simulink model "F2026_ECE597_01_Closed_Loop_Step_Response_PID"  (R2025a)
settings: Solver=VariableStepAuto  StartTime=0.0  StopTime=60.0  RelTol=1e-3
values from neighbouring files (symbols this model uses):
  A = [[-0.59 0.92 0.61 -9.82]; [-0.23 -6.31 4.42 0.19]; [ 0.78 -5.59 -5.92 0]; [0 0 1 0]]    [F2026_ECE597_01_Closed_Loop_Step_Response_PID_Driver.m]
  B = B_w_wind(:,1:2)    [F2026_ECE597_01_Closed_Loop_Step_Response_PID_Driver.m]
  C = [[1 0 0 0]; [0 0 0 1]]    [F2026_ECE597_01_Closed_Loop_Step_Response_PID_Driver.m]
  D = zeros(2, 2)    [F2026_ECE597_01_Closed_Loop_Step_Response_PID_Driver.m]
  delta_airspeed = target_airspeed - airspeed_init    (= 2.1)    [F2026_ECE597_01_Closed_Loop_Step_Response_PID_Driver.m]
  delta_pitch = target_pitch - pitch_init    [F2026_ECE597_01_Closed_Loop_Step_Response_PID_Driver.m]
  elevator_max = deg2rad(20) - elevator_init    [F2026_ECE597_01_Closed_Loop_Step_Response_PID_Driver.m]
  elevator_min = -deg2rad(20) - elevator_init    [F2026_ECE597_01_Closed_Loop_Step_Response_PID_Driver.m]
  G_Airspeed = 1.0    (= 1)    [F2026_ECE597_01_Closed_Loop_Step_Response_PID_Driver.m]
  G_Decoupler = [0.019614 -0.005618; 0.036387 0.501756]    [F2026_ECE597_01_Closed_Loop_Step_Response_PID_Driver.m]
  G_Pitch_Angle = 1.0    (= 1)    [F2026_ECE597_01_Closed_Loop_Step_Response_PID_Driver.m]
  kD_1 = 0.43    [F2026_ECE597_01_Closed_Loop_Step_Response_PID_Driver.m]
  kD_2 = 1.04    [F2026_ECE597_01_Closed_Loop_Step_Response_PID_Driver.m]
  kI_1 = 1.54    [F2026_ECE597_01_Closed_Loop_Step_Response_PID_Driver.m]
  kI_2 = 1.46    [F2026_ECE597_01_Closed_Loop_Step_Response_PID_Driver.m]
  kP_1 = 0.98    [F2026_ECE597_01_Closed_Loop_Step_Response_PID_Driver.m]
  kP_2 = 2.97    [F2026_ECE597_01_Closed_Loop_Step_Response_PID_Driver.m]
  throttle_max = 1.0 - throttle_init    (= 0.56)    [F2026_ECE597_01_Closed_Loop_Step_Response_PID_Driver.m]
  throttle_min = 0.0 - throttle_init    (= -0.44)    [F2026_ECE597_01_Closed_Loop_Step_Response_PID_Driver.m]
libraries: slpidlib x2
settings Model: Creator=gresham2  LastModifiedBy=gresham2

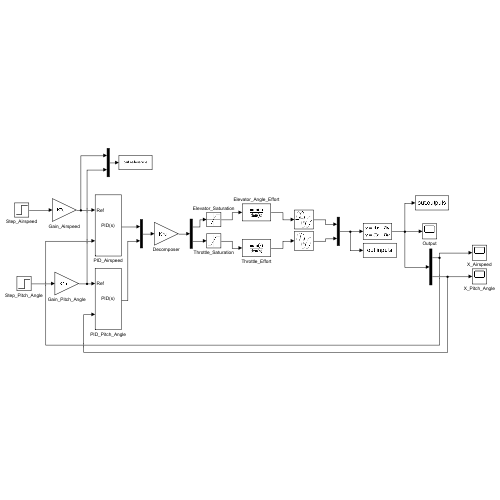
[thumbnail: Simulink's stored preview of the top-level diagram]
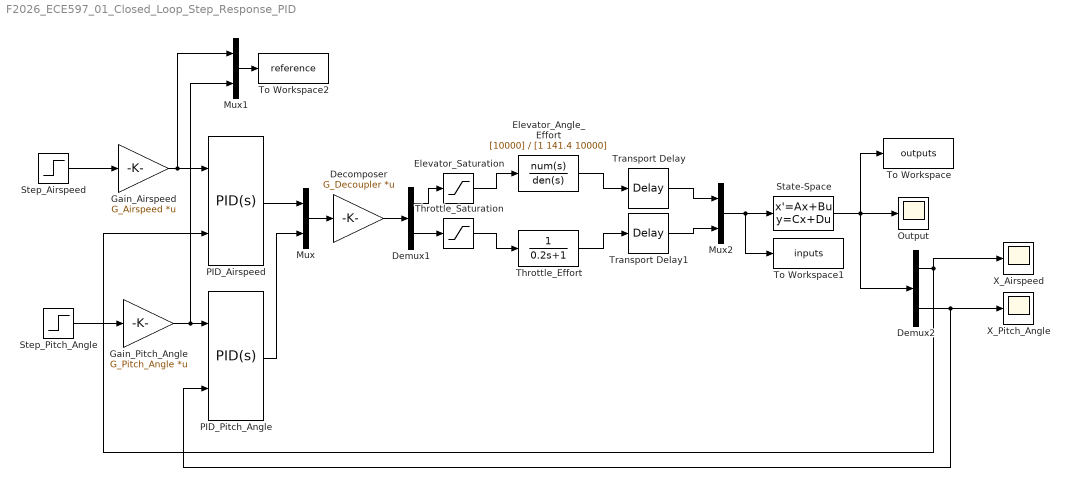
== system F2026_ECE597_01_Closed_Loop_Step_Response_PID ==
  Decomposer : Gain  Gain=G_Decoupler  Multiplication=Matrix(K*u)
  Demux1 : Demux  Outputs=2
  Demux2 : Demux  Outputs=2
  Elevator_Angle_Effort : TransferFcn  Numerator=[10000]  Denominator=[1 141.4 10000]
  Elevator_Saturation : Saturate  UpperLimit=elevator_max  LowerLimit=elevator_min
  Gain_Airspeed : Gain  Gain=G_Airspeed  Multiplication=Matrix(K*u)
  Gain_Pitch_Angle : Gain  Gain=G_Pitch_Angle  Multiplication=Matrix(K*u)
  Mux : Mux  Inputs=2
  Mux1 : Mux  Inputs=2
  Mux2 : Mux  Inputs=2
  Output : Scope
      settings: ActiveDisplayYMinimum=-1  ActiveDisplayYMaximum=1
  PID_Airspeed : slpidlib/PID Controller (2DOF)  Controller=PID  Form=Parallel  TimeDomain=Continuous-time  UseExternalTs=off  SampleTime=-1  IntegratorMethod=Forward Euler  FilterMethod=Forward Euler  ControllerParametersSource=internal  P=kP_1  I=kI_1  UseKiTs=off  D=kD_1  UseExternalDerivativeSource=off  N=100  UseFilter=on  b=1.0  c=0.0  TunerSelectOption=Transfer Function Based (PID Tuner App)  InitialConditionSource=internal  InitialConditionForIntegrator=0  InitialConditionForFilter=0  DifferentiatorICPrevScaledInput=0  ExternalReset=none  TrackingMode=off  Kt=1  LimitOutput=off  SatLimitsSource=internal  UpperSaturationLimit=inf  LowerSaturationLimit=-inf  LinearizeAsGain=on  AntiWindupMode=none  Kb=1  LimitIntegrator=off  UpperIntegratorSaturationLimit=inf  LowerIntegratorSaturationLimit=-inf  POutMin=[]  POutMax=[]  IOutMin=[]  IOutMax=[]  DOutMin=[]  DOutMax=[]  NOutMin=[]  NOutMax=[]  bOutMin=[]  bOutMax=[]  cOutMin=[]  cOutMax=[]  SumOutMin=[]  SumOutMax=[]  SaturationOutMin=[]  SaturationOutMax=[]  PParamMin=[]  PParamMax=[]  IParamMin=[]  IParamMax=[]  DParamMin=[]  DParamMax=[]  NParamMin=[]  NParamMax=[]  bParamMin=[]  bParamMax=[]  cParamMin=[]  cParamMax=[]  KbParamMin=[]  KbParamMax=[]  KtParamMin=[]  KtParamMax=[]  KbOutMin=[]  KbOutMax=[]  KtOutMin=[]  KtOutMax=[]  IntegratorOutMin=[]  IntegratorOutMax=[]  FilterOutMin=[]  FilterOutMax=[]  SumI1OutMin=[]  SumI1OutMax=[]  SumI2OutMin=[]  SumI2OutMax=[]  SumI3OutMin=[]  SumI3OutMax=[]  SumI4OutMin=[]  SumI4OutMax=[]  SumDOutMin=[]  SumDOutMax=[]  Sum1OutMin=[]  Sum1OutMax=[]  Sum2OutMin=[]  Sum2OutMax=[]  Sum3OutMin=[]  Sum3OutMax=[]  DifferentiatorOutMin=[]  DifferentiatorOutMax=[]  FilterDiffOutCoefMin=[]  FilterDiffOutCoefMax=[]  ReciprocalOutMin=[]  ReciprocalOutMax=[]  SumDenOutMin=[]  SumDenOutMax=[]  SumNumOutMin=[]  SumNumOutMax=[]  DivideOutMin=[]  DivideOutMax=[]  UdiffTsProdOutMin=[]  UdiffTsProdOutMax=[]  NTsProdOutMin=[]  NTsProdOutMax=[]  UintegralTsProdOutMin=[]  UintegralTsProdOutMax=[]  UngainTsProdOutMin=[]  UngainTsProdOutMax=[]  ClampingZeroOutDataTypeStr=Inherit: Inherit via back propagation  ClampingZeroOutMin=[]  ClampingZeroOutMax=[]  FilterDenConstantOutDataTypeStr=Inherit: Inherit via back propagation  FilterDenConstantOutMin=[]  FilterDenConstantOutMax=[]  PCopyOutDataTypeStr=Inherit: Inherit via back propagation  PCopyOutMin=[]  PCopyOutMax=[]  NCopyOutDataTypeStr=Inherit: Inherit via back propagation  NCopyOutMin=[]  NCopyOutMax=[]  IntegratorContinuousStateAttributes=''  IntegratorStateMustResolveToSignalObject=off  IntegratorRTWStateStorageClass=Auto  FilterContinuousStateAttributes=''  FilterStateMustResolveToSignalObject=off  FilterRTWStateStorageClass=Auto  ParallelPVariant=InternalParameters  IdealPVariant=Disabled  IVariant=InternalParameters  DVariant=InternalParameters  bVariant=InternalParameters  cVariant=InternalParameters  IntegratorVariant=Continuous  SatVariant=Disabled  AWVariant=Passthrough  PCopyVariant=Disabled  TRVariant=Disabled  FdbkBlocksVariant=Forward  IdealPFdbkVariant=Disabled  SatFdbkVariant=Disabled  DerivativeFilterVariant=ContFilter  NVariant=InternalParameters  NCopyVariant=Disabled  FilterICVariant=InternalICsFilter  IntegratorICVariant=InternalICs  ExternalResetVariant=Disabled  TRSumVariant=Passthrough  SumFdbkVariant=Disabled  SumVariant=Sum_PID  TsampFilterVariant=InternalTs  TsampNgainVariant=Passthrough  TsampIntegralVariant=Disabled_SignalSpec  ExternalSaturationOutDataTypeStr=Inherit: Same as second input  DerivativeSourceVariant=ErrorSignal  PreIntVariant=InternalPreInt
  PID_Pitch_Angle : slpidlib/PID Controller (2DOF)  Controller=PID  Form=Parallel  TimeDomain=Continuous-time  UseExternalTs=off  SampleTime=-1  IntegratorMethod=Forward Euler  FilterMethod=Forward Euler  ControllerParametersSource=internal  P=kP_2  I=kI_2  UseKiTs=off  D=kD_2  UseExternalDerivativeSource=off  N=100  UseFilter=on  b=1.0  c=0.0  TunerSelectOption=Transfer Function Based (PID Tuner App)  InitialConditionSource=internal  InitialConditionForIntegrator=0  InitialConditionForFilter=0  DifferentiatorICPrevScaledInput=0  ExternalReset=none  TrackingMode=off  Kt=1  LimitOutput=off  SatLimitsSource=internal  UpperSaturationLimit=inf  LowerSaturationLimit=-inf  LinearizeAsGain=on  AntiWindupMode=none  Kb=1  LimitIntegrator=off  UpperIntegratorSaturationLimit=inf  LowerIntegratorSaturationLimit=-inf  POutMin=[]  POutMax=[]  IOutMin=[]  IOutMax=[]  DOutMin=[]  DOutMax=[]  NOutMin=[]  NOutMax=[]  bOutMin=[]  bOutMax=[]  cOutMin=[]  cOutMax=[]  SumOutMin=[]  SumOutMax=[]  SaturationOutMin=[]  SaturationOutMax=[]  PParamMin=[]  PParamMax=[]  IParamMin=[]  IParamMax=[]  DParamMin=[]  DParamMax=[]  NParamMin=[]  NParamMax=[]  bParamMin=[]  bParamMax=[]  cParamMin=[]  cParamMax=[]  KbParamMin=[]  KbParamMax=[]  KtParamMin=[]  KtParamMax=[]  KbOutMin=[]  KbOutMax=[]  KtOutMin=[]  KtOutMax=[]  IntegratorOutMin=[]  IntegratorOutMax=[]  FilterOutMin=[]  FilterOutMax=[]  SumI1OutMin=[]  SumI1OutMax=[]  SumI2OutMin=[]  SumI2OutMax=[]  SumI3OutMin=[]  SumI3OutMax=[]  SumI4OutMin=[]  SumI4OutMax=[]  SumDOutMin=[]  SumDOutMax=[]  Sum1OutMin=[]  Sum1OutMax=[]  Sum2OutMin=[]  Sum2OutMax=[]  Sum3OutMin=[]  Sum3OutMax=[]  DifferentiatorOutMin=[]  DifferentiatorOutMax=[]  FilterDiffOutCoefMin=[]  FilterDiffOutCoefMax=[]  ReciprocalOutMin=[]  ReciprocalOutMax=[]  SumDenOutMin=[]  SumDenOutMax=[]  SumNumOutMin=[]  SumNumOutMax=[]  DivideOutMin=[]  DivideOutMax=[]  UdiffTsProdOutMin=[]  UdiffTsProdOutMax=[]  NTsProdOutMin=[]  NTsProdOutMax=[]  UintegralTsProdOutMin=[]  UintegralTsProdOutMax=[]  UngainTsProdOutMin=[]  UngainTsProdOutMax=[]  ClampingZeroOutDataTypeStr=Inherit: Inherit via back propagation  ClampingZeroOutMin=[]  ClampingZeroOutMax=[]  FilterDenConstantOutDataTypeStr=Inherit: Inherit via back propagation  FilterDenConstantOutMin=[]  FilterDenConstantOutMax=[]  PCopyOutDataTypeStr=Inherit: Inherit via back propagation  PCopyOutMin=[]  PCopyOutMax=[]  NCopyOutDataTypeStr=Inherit: Inherit via back propagation  NCopyOutMin=[]  NCopyOutMax=[]  IntegratorContinuousStateAttributes=''  IntegratorStateMustResolveToSignalObject=off  IntegratorRTWStateStorageClass=Auto  FilterContinuousStateAttributes=''  FilterStateMustResolveToSignalObject=off  FilterRTWStateStorageClass=Auto  ParallelPVariant=InternalParameters  IdealPVariant=Disabled  IVariant=InternalParameters  DVariant=InternalParameters  bVariant=InternalParameters  cVariant=InternalParameters  IntegratorVariant=Continuous  SatVariant=Disabled  AWVariant=Passthrough  PCopyVariant=Disabled  TRVariant=Disabled  FdbkBlocksVariant=Forward  IdealPFdbkVariant=Disabled  SatFdbkVariant=Disabled  DerivativeFilterVariant=ContFilter  NVariant=InternalParameters  NCopyVariant=Disabled  FilterICVariant=InternalICsFilter  IntegratorICVariant=InternalICs  ExternalResetVariant=Disabled  TRSumVariant=Passthrough  SumFdbkVariant=Disabled  SumVariant=Sum_PID  TsampFilterVariant=InternalTs  TsampNgainVariant=Passthrough  TsampIntegralVariant=Disabled_SignalSpec  ExternalSaturationOutDataTypeStr=Inherit: Same as second input  DerivativeSourceVariant=ErrorSignal  PreIntVariant=InternalPreInt
  State-Space : StateSpace  A=A  B=B  C=C  D=D  InitialCondition=0
  Step_Airspeed : Step  After=delta_airspeed  SampleTime=0
  Step_Pitch_Angle : Step  After=delta_pitch  SampleTime=0
  Throttle_Effort : TransferFcn  Denominator=[0.2 1]
  Throttle_Saturation : Saturate  UpperLimit=throttle_max  LowerLimit=throttle_min
  To Workspace : ToWorkspace  VariableName=outputs  SaveFormat=Timeseries  SampleTime=-1
  To Workspace1 : ToWorkspace  VariableName=inputs  SaveFormat=Timeseries  SampleTime=-1
  To Workspace2 : ToWorkspace  VariableName=reference  SaveFormat=Timeseries  SampleTime=-1
  Transport Delay : TransportDelay  DelayTime=0.07
  Transport Delay1 : TransportDelay  DelayTime=0.05
  X_Airspeed : Scope
      settings: ActiveDisplayYMinimum=-1  ActiveDisplayYMaximum=1  DataLoggingVariableName=ScopeData4
  X_Pitch_Angle : Scope
      settings: ActiveDisplayYMinimum=-1  ActiveDisplayYMaximum=1  DataLoggingVariableName=ScopeData3
  wires:
  State-Space/1 -> To Workspace/1, Output/1, Demux2/1
  Demux2/1 -> X_Airspeed/1, PID_Airspeed/2
  Demux2/2 -> X_Pitch_Angle/1, PID_Pitch_Angle/2
  Step_Airspeed/1 -> Gain_Airspeed/1
  Gain_Airspeed/1 -> Mux1/1, PID_Airspeed/1
  Gain_Pitch_Angle/1 -> Mux1/2, PID_Pitch_Angle/1
  Step_Pitch_Angle/1 -> Gain_Pitch_Angle/1
  Mux/1 -> Decomposer/1
  PID_Airspeed/1 -> Mux/1
  PID_Pitch_Angle/1 -> Mux/2
  Mux1/1 -> To Workspace2/1
  Decomposer/1 -> Demux1/1
  Demux1/2 -> Throttle_Saturation/1
  Demux1/1 -> Elevator_Saturation/1
  Mux2/1 -> To Workspace1/1, State-Space/1
  Elevator_Angle_Effort/1 -> Transport Delay/1
  Throttle_Effort/1 -> Transport Delay1/1
  Elevator_Saturation/1 -> Elevator_Angle_Effort/1
  Throttle_Saturation/1 -> Throttle_Effort/1
  Transport Delay/1 -> Mux2/1
  Transport Delay1/1 -> Mux2/2
